simulink model "kundur_sync"  (R2023b)
settings: Solver=ode23tb  StartTime=0.0  StopTime=200  MaxStep=1/60  RelTol=1e-3
InitFcn:
  | SolarInverter_Params();
values from neighbouring files (symbols this model uses):
  Fnom = 60    [SolarInverter_Params.m]
  Pnom = 900e6    (= 900000000)    [SolarInverter_Params.m]
  reec_dbd1 = -0.1    [SolarInverter_Params.m]
  reec_dbd2 = 0.1    [SolarInverter_Params.m]
  reec_dPmax = 0.1    [SolarInverter_Params.m]
  reec_dPmin = -0.1    [SolarInverter_Params.m]
  reec_Imax = 1    [SolarInverter_Params.m]
  reec_Iqhl = 1.0    (= 1)    [SolarInverter_Params.m]
  reec_Iqll = -0.4    [SolarInverter_Params.m]
  reec_Kqi = 0.0    (= 0)    [SolarInverter_Params.m]
  reec_Kqp = 0    [SolarInverter_Params.m]
  reec_Kvi = 0.0    (= 0)    [SolarInverter_Params.m]
  reec_Kvp = 0.1    [SolarInverter_Params.m]
  reec_Pmax = 1.0    (= 1)    [SolarInverter_Params.m]
  reec_Pmin = 0    [SolarInverter_Params.m]
  reec_Qmax = 0.435    [SolarInverter_Params.m]
  reec_Qmin = -0.435    [SolarInverter_Params.m]
  reec_Tiq = 0.02    [SolarInverter_Params.m]
  reec_Tp = 0.02    [SolarInverter_Params.m]
  reec_Tpord = 0.1    [SolarInverter_Params.m]
  reec_Trv = 0.01    [SolarInverter_Params.m]
  reec_Vdip = 0.9    [SolarInverter_Params.m]
  reec_Vmax = 1.10    (= 1.1)    [SolarInverter_Params.m]
  reec_Vmin = 0.9    [SolarInverter_Params.m]
  reec_Vup = 1.15    [SolarInverter_Params.m]
  regc_Brkpt = 0.9    [SolarInverter_Params.m]
  regc_Iolim = -1.2    [SolarInverter_Params.m]
  regc_Iqrmax = 999.9    [SolarInverter_Params.m]
  regc_Iqrmin = -999.9    [SolarInverter_Params.m]
  regc_Ivpnt0 = 0.4    [SolarInverter_Params.m]
  regc_Ivpnt1 = 0.8    [SolarInverter_Params.m]
  regc_Khv = 0.0    (= 0)    [SolarInverter_Params.m]
  regc_Lvpl1 = 1.0    (= 1)    [SolarInverter_Params.m]
  regc_Lvplsw = 0    [SolarInverter_Params.m]
  regc_rrpwr = 10    [SolarInverter_Params.m]
  regc_Tfltr = 0.02    [SolarInverter_Params.m]
  regc_Tg = 0.1    [SolarInverter_Params.m]
  regc_Volim = 1.1    [SolarInverter_Params.m]
  regc_Zerox = 0.5    [SolarInverter_Params.m]
  repc_db1 = 0    [SolarInverter_Params.m]
  repc_Ddn = 20    [SolarInverter_Params.m]
  repc_Dup = 0    [SolarInverter_Params.m]
  repc_emax = 999    [SolarInverter_Params.m]
  repc_emin = -999    [SolarInverter_Params.m]
  repc_fdbd1 = 0.01*0    (= 0)    [SolarInverter_Params.m]
  repc_fdbd2 = -0.01*0    (= 0)    [SolarInverter_Params.m]
  repc_femax = 999    [SolarInverter_Params.m]
  repc_femin = -999    [SolarInverter_Params.m]
  repc_Kc = 0.05    [SolarInverter_Params.m]
  repc_Ki = 1.8    [SolarInverter_Params.m]
  repc_Kig = 0.5    [SolarInverter_Params.m]
  repc_Kp = 0.6    [SolarInverter_Params.m]
  repc_Kpg = 0.1    [SolarInverter_Params.m]
  repc_Pmax = 1    [SolarInverter_Params.m]
  repc_Pmin = 0    [SolarInverter_Params.m]
  repc_Qmax = 0.435    [SolarInverter_Params.m]
  repc_Qmin = -0.435    [SolarInverter_Params.m]
  repc_Rc = 0    [SolarInverter_Params.m]
  repc_Tfltr = 0.02    [SolarInverter_Params.m]
  repc_Tft = 0.5    [SolarInverter_Params.m]
  repc_Tfv = 0.8    [SolarInverter_Params.m]
  repc_Tlag = 0.2    [SolarInverter_Params.m]
  repc_Tp = 0.25    [SolarInverter_Params.m]
  repc_Vfrz = 0.7    [SolarInverter_Params.m]
  repc_Xc = 0    [SolarInverter_Params.m]
  Vnom = 230e3    (= 230000)    [SolarInverter_Params.m]
undefined symbols (not defined in the file or in its folder): D1, Delta, gcbh, j, k_fault, k_pulse, sps_rtmsupport
libraries: powerlib_extras x24, simulink x13, spsLoadFlowBusLib x12, spsThreePhaseVIMeasurementLib x11, spsThreePhasePISectionLineLib x8, spsThreePhaseTransformerTwoWindingsLib x5, spsThreePhaseParallelRLCLoadLib x4, spsSynchronousMachinepuStandardLib x4, spsExcitationSystemLib x4, spsSteamTurbineandGovernorLib x4, spsGenericPowerSystemStabilizerLib x4, spsControlledCurrentSourceLib x2
(part 1 of 3)
settings Model: Creator=jlesage  LastModifiedBy=shura
settings SolverCC: ZeroCrossAlgorithm=Adaptive
settings DataIOCC: InitialState=getstatestruct(opreport)  SaveOutput=off  SignalLogging=off  DSMLogging=off  SaveTime=off  ReturnWorkspaceOutputs=off
settings DebuggingCC: IgnoredZcDiagnostic=none
settings ModelReferenceCC: EnableRefExpFcnMdlSchedulingChecks=on
settings SFSimCC: CustomCodeUndefinedFunction=UseInterfaceOnly
settings SimscapeCC: SimscapeNormalizeSystem=off

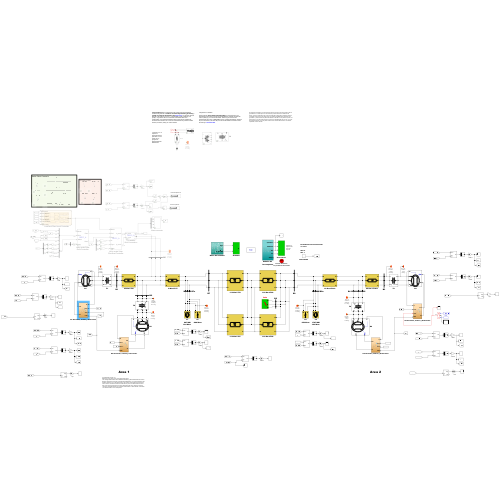
[thumbnail: Simulink's stored preview of the top-level diagram]
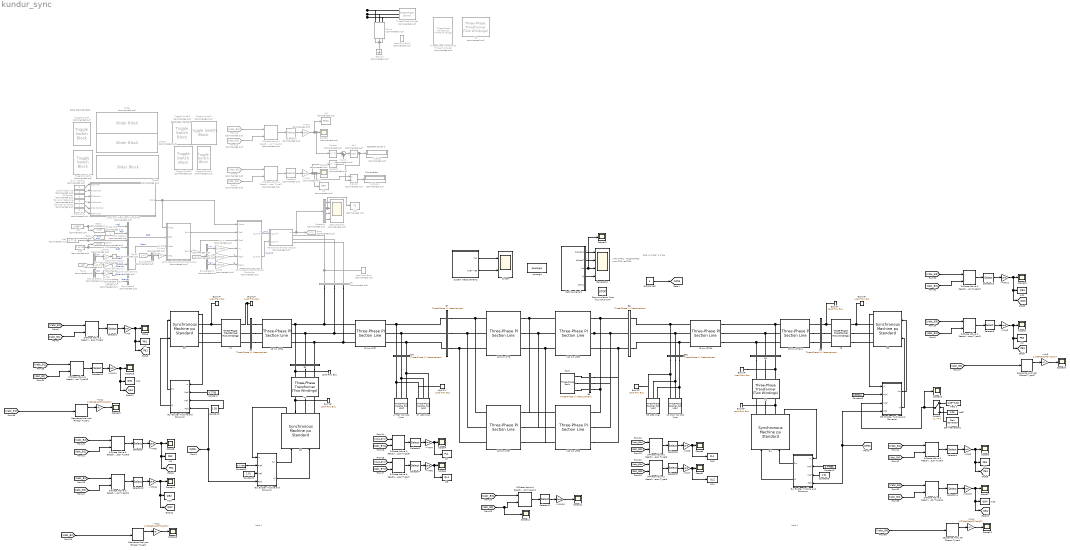
== system kundur_sync ==
  note: Solar Plant Controls
  note: Secondary Controls
  note: yellow=G1,
      | magenta=G2,
      | cyan=G3,
      | red=G4
  note: Area 2
  note: Area 1
  note: PSS: 0 = OFF, 1 = ON
  note: Power factor
  note: Apparent power S
  ->MW{,2..8,10..14} (13 alike) : Gain  Gain=1e-6  SaturateOnIntegerOverflow=on  OutDataTypeStr=Inherit: Same as input  ParamDataTypeStr=Inherit: Same as input
  ->MW1 : Gain  Commented=on  Gain=1e-6  SaturateOnIntegerOverflow=on  OutDataTypeStr=Inherit: Same as input  ParamDataTypeStr=Inherit: Same as input
  ->MW9 : Gain  Commented=on  Gain=1e-6  SaturateOnIntegerOverflow=on  OutDataTypeStr=Inherit: Same as input  ParamDataTypeStr=Inherit: Same as input
  ->pu{1..4} (4 alike) : Gain  Gain=1/(230e3/sqrt(3)*sqrt(2))  SaturateOnIntegerOverflow=on  OutDataTypeStr=Inherit: Same as input  ParamDataTypeStr=Inherit: Same as input
  10 Km LT67 : spsThreePhasePISectionLineLib/Three-Phase PI Section Line  LConnTagsString=a|b|c  RConnTagsString=A|B|C  Length=10  Frequency=60  Resistances=[0.0001*529 1.61]  Inductances=[0.001*529/(377) 0.0061]  Capacitances=[0.00175/529/(377) 5.2489e-9]
  10 Km LT910 : spsThreePhasePISectionLineLib/Three-Phase PI Section Line  LConnTagsString=a|b|c  RConnTagsString=A|B|C  Length=10  Frequency=60  Resistances=[0.0001*529 1.61]  Inductances=[0.001*529/(377) 0.0061]  Capacitances=[0.00175/529/(377) 5.2489e-9]
  110 Km LT{78,87,89,98} (4 alike) : spsThreePhasePISectionLineLib/Three-Phase PI Section Line  LConnTagsString=a|b|c  RConnTagsString=A|B|C  Length=110  Frequency=60  Resistances=[0.0001*529 1.61]  Inductances=[0.001*529/(377) 0.0061]  Capacitances=[0.00175/529/(377) 5.2489e-9]
  25 Km LT1011 : spsThreePhasePISectionLineLib/Three-Phase PI Section Line  LConnTagsString=a|b|c  RConnTagsString=A|B|C  Length=25  Frequency=60  Resistances=[0.0001*529 1.61]  Inductances=[0.001*529/(377) 0.0061]  Capacitances=[0.00175/529/(377) 5.2489e-9]
  25 Km LT56 : spsThreePhasePISectionLineLib/Three-Phase PI Section Line  LConnTagsString=a|b|c  RConnTagsString=A|B|C  Length=25  Frequency=60  Resistances=[0.0001*529 1.61]  Inductances=[0.001*529/(377) 0.0061]  Capacitances=[0.00175/529/(377) 5.2489e-9]
  3-Phase Active & Reactive Power (Phasor Type){1,3..9,11..15} (13 alike) : powerlib_extras/Phasor Library/3-Phase Active & Reactive Power (Phasor Type)
  3-Phase Active & Reactive Power (Phasor Type)10 : powerlib_extras/Phasor Library/3-Phase Active & Reactive Power (Phasor Type)  Commented=on
  3-Phase Active & Reactive Power (Phasor Type)2 : powerlib_extras/Phasor Library/3-Phase Active & Reactive Power (Phasor Type)  Commented=on
  B1 : spsThreePhaseVIMeasurementLib/Three-Phase V-I Measurement  VoltageMeasurement=phase-to-ground  SetLabelV=on  LabelV=Vabc_B1  Vpu=off  VpuLL=off  CurrentMeasurement=yes  SetLabelI=on  LabelI=Iabc_B1  Ipu=off  Pbase=100e6  Vbase=500e3  OutputType=Complex  PhasorSimulation=on  PSBequivalent=0
  B2 : spsThreePhaseVIMeasurementLib/Three-Phase V-I Measurement  VoltageMeasurement=phase-to-ground  SetLabelV=on  LabelV=Vabc_B2  Vpu=off  VpuLL=off  CurrentMeasurement=yes  SetLabelI=on  LabelI=Iabc_B2  Ipu=off  Pbase=100e6  Vbase=500e3  OutputType=Complex  PhasorSimulation=on  PSBequivalent=0
  B3 : spsThreePhaseVIMeasurementLib/Three-Phase V-I Measurement  VoltageMeasurement=phase-to-ground  SetLabelV=on  LabelV=Vabc_B3  Vpu=off  VpuLL=off  CurrentMeasurement=yes  SetLabelI=on  LabelI=Iabc_B3  Ipu=off  Pbase=100e6  Vbase=500e3  OutputType=Complex  PhasorSimulation=on  PSBequivalent=0
  B4 : spsThreePhaseVIMeasurementLib/Three-Phase V-I Measurement  VoltageMeasurement=phase-to-ground  SetLabelV=on  LabelV=Vabc_B4  Vpu=off  VpuLL=off  CurrentMeasurement=yes  SetLabelI=on  LabelI=Iabc_B4  Ipu=off  Pbase=100e6  Vbase=500e3  OutputType=Complex  PhasorSimulation=on  PSBequivalent=0
  B5 : spsThreePhaseVIMeasurementLib/Three-Phase V-I Measurement  Commented=on  VoltageMeasurement=phase-to-ground  SetLabelV=on  LabelV=Vabc_B5  Vpu=off  VpuLL=off  CurrentMeasurement=yes  SetLabelI=on  LabelI=Iabc_B5  Ipu=off  Pbase=100e6  Vbase=500e3  OutputType=Complex  PhasorSimulation=on  PSBequivalent=0
  B6 : spsThreePhaseVIMeasurementLib/Three-Phase V-I Measurement  VoltageMeasurement=phase-to-ground  SetLabelV=on  LabelV=Vabc_B8  Vpu=off  VpuLL=off  CurrentMeasurement=yes  SetLabelI=on  LabelI=Iabc_B8  Ipu=off  Pbase=100e6  Vbase=500e3  OutputType=Complex  PhasorSimulation=on  PSBequivalent=0
  B7 : spsThreePhaseVIMeasurementLib/Three-Phase V-I Measurement  VoltageMeasurement=phase-to-ground  SetLabelV=on  LabelV=Vabc_B7  Vpu=off  VpuLL=off  CurrentMeasurement=yes  SetLabelI=on  LabelI=Iabc_B7  Ipu=off  Pbase=100e6  Vbase=500e3  OutputType=Complex  PhasorSimulation=on  PSBequivalent=0
  B7c : spsThreePhaseVIMeasurementLib/Three-Phase V-I Measurement  VoltageMeasurement=phase-to-ground  SetLabelV=on  LabelV=Vabc_B7c  Vpu=off  VpuLL=off  CurrentMeasurement=yes  SetLabelI=on  LabelI=Iabc_B7c  Ipu=off  Pbase=100e6  Vbase=500e3  OutputType=Complex  PhasorSimulation=on  PSBequivalent=0
  B9 : spsThreePhaseVIMeasurementLib/Three-Phase V-I Measurement  VoltageMeasurement=phase-to-ground  SetLabelV=on  LabelV=Vabc_B9  Vpu=off  VpuLL=off  CurrentMeasurement=yes  SetLabelI=on  LabelI=Iabc_B9  Ipu=off  Pbase=100e6  Vbase=500e3  OutputType=Complex  PhasorSimulation=on  PSBequivalent=0
  B9c : spsThreePhaseVIMeasurementLib/Three-Phase V-I Measurement  VoltageMeasurement=phase-to-ground  SetLabelV=on  LabelV=Vabc_B9c  Vpu=off  VpuLL=off  CurrentMeasurement=yes  SetLabelI=on  LabelI=Iabc_B9c  Ipu=off  Pbase=100e6  Vbase=500e3  OutputType=Complex  PhasorSimulation=on  PSBequivalent=0
  Bus Creator1 : BusCreator  Commented=on  Inputs=4
  Bus Creator2 : BusCreator  Commented=on  Inputs=4
  Bus Selector1 : BusSelector  Commented=on  OutputSignals=V,P,Q
  Bus Selector2 : BusSelector  Commented=on  OutputSignals=F,P,Q
  Bus Selector3 : BusSelector  Commented=on  OutputSignals=V
  Bus*13* : spsLoadFlowBusLib/Load Flow Bus  LConnTagsString=a  Phases=single  Connectors=on one side  ID=Bus*13*  Vbase=230000  Vref=1  Vangle=0  VLF=1.007  VLFb=1  VLFc=1  angleLF=43.46  angleLFb=0  angleLFc=0
  Bus*14* : spsLoadFlowBusLib/Load Flow Bus  LConnTagsString=a  Phases=single  Connectors=on one side  ID=Bus*14*  Vbase=20000  Vref=1.03  Vangle=20.2  VLF=1.03  VLFb=1  VLFc=1  angleLF=19.92  angleLFb=0  angleLFc=0
  Bus*16* : spsLoadFlowBusLib/Load Flow Bus  LConnTagsString=a  Phases=single  Connectors=on one side  ID=Bus*16*  Vbase=20000  Vref=1.01  Vangle=10.5  VLF=1.01  VLFb=1  VLFc=1  angleLF=10.17  angleLFb=0  angleLFc=0
  Bus*17* : spsLoadFlowBusLib/Load Flow Bus  LConnTagsString=a  Phases=single  Connectors=on one side  ID=Bus*17*  Vbase=230000  Vref=1  Vangle=0  VLF=1.009  VLFb=1  VLFc=1  angleLF=16.59  angleLFb=0  angleLFc=0
  Bus*18* : spsLoadFlowBusLib/Load Flow Bus  LConnTagsString=a  Phases=single  Connectors=on one side  ID=Bus*18*  Vbase=20000  Vref=1.03  Vangle=-6.8  VLF=1.03  VLFb=1  VLFc=1  angleLF=-6.8  angleLFb=0  angleLFc=0
  Bus*19* : spsLoadFlowBusLib/Load Flow Bus  LConnTagsString=a  Phases=single  Connectors=on one side  ID=Bus*19*  Vbase=230000  Vref=1  Vangle=0  VLF=0.9863  VLFb=1  VLFc=1  angleLF=6.317  angleLFb=0  angleLFc=0
  Bus*20* : spsLoadFlowBusLib/Load Flow Bus  LConnTagsString=a  Phases=single  Connectors=on one side  ID=Bus*20*  Vbase=20000  Vref=1.01  Vangle=-17  VLF=1.01  VLFb=1  VLFc=1  angleLF=-16.96  angleLFb=0  angleLFc=0
  Bus*21* : spsLoadFlowBusLib/Load Flow Bus  LConnTagsString=a  Phases=single  Connectors=on one side  ID=Bus*21*  Vbase=230000  Vref=1  Vangle=0  VLF=0.9654  VLFb=1  VLFc=1  angleLF=25.05  angleLFb=0  angleLFc=0
  Bus*22* : spsLoadFlowBusLib/Load Flow Bus  LConnTagsString=a  Phases=single  Connectors=on one side  ID=Bus*22*  Vbase=230000  Vref=1  Vangle=0  VLF=0.9765  VLFb=1  VLFc=1  angleLF=-2.038  angleLFb=0  angleLFc=0
  C7 -200 Mvar : spsThreePhaseParallelRLCLoadLib/Three-Phase Parallel RLC Load  LConnTagsString=A|B|C  Configuration=Y (grounded)  NominalVoltage=(230000)*0.965432  Vabc=[1e3 1e3 1e3]  Vabcp=[1e3 1e3 1e3]  NominalFrequency=60  UnbalancedPower=off  ActivePower=0  InductivePower=0  CapacitivePower=200000000  Pabc=[10e3 9e3 11e3]  QLabc=[100 90 110]  QCabc=[100 90 110]  Pabcp=[10e3 9e3 11e3]  QLabcp=[100 90 110]  QCabcp=[100 90 110]  Measurements=None  LoadType=constant PQ
  C9 -350 Mvar : spsThreePhaseParallelRLCLoadLib/Three-Phase Parallel RLC Load  LConnTagsString=A|B|C  Configuration=Y (grounded)  NominalVoltage=(230000)*0.976525  Vabc=[1e3 1e3 1e3]  Vabcp=[1e3 1e3 1e3]  NominalFrequency=60  UnbalancedPower=off  ActivePower=0  InductivePower=0  CapacitivePower=350000000  Pabc=[10e3 9e3 11e3]  QLabc=[100 90 110]  QCabc=[100 90 110]  Pabcp=[10e3 9e3 11e3]  QLabcp=[100 90 110]  QCabcp=[100 90 110]  Measurements=None  LoadType=constant PQ
  Constant : Constant  Value=0.7793
  Constant1 : Constant  Value=1.03
  Constant13 : Constant  Commented=on
  Constant14 : Constant  Commented=on  Value=0
  Constant2 : Constant  Value=0.77941
  Constant3 : Constant  Value=1.01
  Constant5 : Constant  Value=0.80012
  Constant6 : Constant  Value=1.01
  Constant7 : Constant  Value=0.77936
  Coordinated V/Q : Constant  Commented=on
  System measurements : Subsystem
  Stop simulation (loss of synchronism) : Stop
  Display : Display  Commented=on
  Display1 : Display  Commented=on
  Fault : spsThreePhaseFaultLib/Three-Phase Fault  InitialStates=0  FaultA=on  FaultB=on  FaultC=on  GroundFault=on  SwitchTimes=[150 150+12/60]*k_fault  External=off  SwitchStatus=NaN  FaultResistance=0.1  GroundResistance=0.1  SnubberResistance=inf  SnubberCapacitance=0  Measurements=None
  From : From  Commented=on  GotoTag=m
  From1 : From  Commented=on  GotoTag=m
  From2 : From  Commented=on  GotoTag=m
  From23 : From  Commented=on  GotoTag=Iabc_B5  TagVisibility=global
      settings: CloseFcn=tagdialog Close
  From24 : From  Commented=on  GotoTag=Vabc_B5  TagVisibility=global
      settings: CloseFcn=tagdialog Close
  From7 : From  Commented=on  GotoTag=Iabc_B5  TagVisibility=global
      settings: CloseFcn=tagdialog Close
  From8 : From  Commented=on  GotoTag=Vabc_B5  TagVisibility=global
      settings: CloseFcn=tagdialog Close
  G1 : spsSynchronousMachinepuStandardLib/Synchronous Machine pu Standard  PresetModel=No  MechanicalLoad=Mechanical power Pm  ShowDetailedParameters=on  RotorType=Round  Units=per unit standard parameters  MeasurementBus=off  NominalParameters=[900E6 20E3 60]  Reactances1=[ 1.8, 0.3, 0.25, 1.7, 0.55, 0.25, 0.2 ]  Reactances2=[2.24 0.17 0.12 1.02 0.13 0.08]  dAxisTimeConstants=Open-circuit  qAxisTimeConstants=Open-circuit  TimeConstants1="[ 4.4849  0.0681  0.1  ]"  TimeConstants2=[ 8.0, 0.03, 0.4, 0.05 ]  TimeConstants3="[  4.49  0.0681  0.0513  ]"  TimeConstants4=[ 8.0, 0.03, 0.3371, 0.0295 ]  TimeConstants5=[ 1.01, 0.053, 0.1 ]  TimeConstants6=[ 1.3201, 0.023, 1.0, 0.07 ]  TimeConstants7=[0.012 0.003 0.003]  TimeConstants8=[ 1.3201, 0.0231, 0.3371, 0.0295 ]  StatorResistance=0.0025  Mechanical=[6.5 0 1]  PolePairs=20  InitialConditions=[0 -26.7419 0.779382 0.779382 0.779382 5.5866 -114.413 125.587 1.9356]  SetSaturation=off  Saturation=[0.6404,0.7127,0.8441,0.9214,0.9956,1.082,1.19,1.316,1.457;0.7,0.7698,0.8872,0.9466,0.9969,1.046,1.1,1.151,1.201]  LoadFlowParameters=[1 700000000 0 0 0]  TsPowergui=0  TsBlock=-1  IterativeModel=Trapezoidal non iterative  IterativeDiscreteModel=Trapezoidal non iterative  BusType=PV  Pref=700000000  Qref=0  Qmin=-Inf  Qmax=Inf  PLF=0  QLF=0
  "G1: Exciter, Turbine and Governor" : Subsystem
  G2 : spsSynchronousMachinepuStandardLib/Synchronous Machine pu Standard  PresetModel=No  MechanicalLoad=Mechanical power Pm  ShowDetailedParameters=on  RotorType=Round  Units=per unit standard parameters  MeasurementBus=off  NominalParameters=[900E6 20E3 60]  Reactances1=[ 1.8, 0.3, 0.25, 1.7, 0.55, 0.25, 0.2 ]  Reactances2=[2.24 0.17 0.12 1.02 0.13 0.08]  dAxisTimeConstants=Open-circuit  qAxisTimeConstants=Open-circuit  TimeConstants1="[ 4.4849  0.0681  0.1  ]"  TimeConstants2=[ 8.0, 0.03, 0.4, 0.05 ]  TimeConstants3="[  4.49  0.0681  0.0513  ]"  TimeConstants4=[ 8.0, 0.03, 0.3371, 0.0295 ]  TimeConstants5=[ 1.01, 0.053, 0.1 ]  TimeConstants6=[ 1.3201, 0.023, 1.0, 0.07 ]  TimeConstants7=[0.012 0.003 0.003]  TimeConstants8=[ 1.3201, 0.0231, 0.3371, 0.0295 ]  StatorResistance=0.0025  Mechanical=[6.5 0 1]  PolePairs=20  InitialConditions=[0 -37.2189 0.807096 0.807096 0.807096 -7.24574 -127.246 112.754 2.00287]  SetSaturation=off  Saturation=[0.6404,0.7127,0.8441,0.9214,0.9956,1.082,1.19,1.316,1.457;0.7,0.7698,0.8872,0.9466,0.9969,1.046,1.1,1.151,1.201]  LoadFlowParameters=[1 700000000 0 0 0]  TsPowergui=0  TsBlock=-1  IterativeModel=Trapezoidal non iterative  IterativeDiscreteModel=Trapezoidal non iterative  BusType=PV  Pref=700000000  Qref=0  Qmin=-Inf  Qmax=Inf  PLF=0  QLF=0
  "G2: Exciter, Turbine and Governor" : Subsystem
  G3 : spsSynchronousMachinepuStandardLib/Synchronous Machine pu Standard  PresetModel=No  MechanicalLoad=Mechanical power Pm  ShowDetailedParameters=on  RotorType=Round  Units=per unit standard parameters  MeasurementBus=off  NominalParameters=[900E6 20E3 60]  Reactances1=[ 1.8, 0.3, 0.25, 1.7, 0.55, 0.25, 0.2 ]  Reactances2=[2.24 0.17 0.12 1.02 0.13 0.08]  dAxisTimeConstants=Open-circuit  qAxisTimeConstants=Open-circuit  TimeConstants1="[ 4.4849  0.0681  0.1  ]"  TimeConstants2=[ 8.0, 0.03, 0.4, 0.05 ]  TimeConstants3="[  4.49  0.0681  0.0513  ]"  TimeConstants4=[ 8.0, 0.03, 0.3371, 0.0295 ]  TimeConstants5=[ 1.01, 0.053, 0.1 ]  TimeConstants6=[ 1.3201, 0.023, 1.0, 0.07 ]  TimeConstants7=[0.012 0.003 0.003]  TimeConstants8=[ 1.3201, 0.0231, 0.3371, 0.0295 ]  StatorResistance=0.0025  Mechanical=[6.175 0 1]  PolePairs=20  InitialConditions=[0 -52.3113 0.79634 0.79634 0.79634 -20.0073 -140.007 99.9927 1.94741]  SetSaturation=off  Saturation=[0.6404,0.7127,0.8441,0.9214,0.9956,1.082,1.19,1.316,1.457;0.7,0.7698,0.8872,0.9466,0.9969,1.046,1.1,1.151,1.201]  LoadFlowParameters=[2 719000000 0 -6.8 0]  TsPowergui=0  TsBlock=-1  IterativeModel=Trapezoidal non iterative  IterativeDiscreteModel=Trapezoidal non iterative  BusType=swing  Pref=Inf  Qref=0  Qmin=-Inf  Qmax=Inf  PLF=0  QLF=0
  "G3: Exciter, Turbine and Governor" : Subsystem
  G4 : spsSynchronousMachinepuStandardLib/Synchronous Machine pu Standard  PresetModel=No  MechanicalLoad=Mechanical power Pm  ShowDetailedParameters=on  RotorType=Round  Units=per unit standard parameters  MeasurementBus=off  NominalParameters=[900E6 20E3 60]  Reactances1=[ 1.8, 0.3, 0.25, 1.7, 0.55, 0.25, 0.2 ]  Reactances2=[2.24 0.17 0.12 1.02 0.13 0.08]  dAxisTimeConstants=Open-circuit  qAxisTimeConstants=Open-circuit  TimeConstants1="[ 4.4849  0.0681  0.1  ]"  TimeConstants2=[ 8.0, 0.03, 0.4, 0.05 ]  TimeConstants3="[  4.49  0.0681  0.0513  ]"  TimeConstants4=[ 8.0, 0.03, 0.3371, 0.0295 ]  TimeConstants5=[ 1.01, 0.053, 0.1 ]  TimeConstants6=[ 1.3201, 0.023, 1.0, 0.07 ]  TimeConstants7=[0.012 0.003 0.003]  TimeConstants8=[ 1.3201, 0.0231, 0.3371, 0.0295 ]  StatorResistance=0.0025  Mechanical=[6.175 0 1]  PolePairs=20  InitialConditions=[0 -62.9983 0.796384 0.796384 0.796384 -31.7259 -151.726 88.2741 1.95328]  SetSaturation=off  Saturation=[0.6404,0.7127,0.8441,0.9214,0.9956,1.082,1.19,1.316,1.457;0.7,0.7698,0.8872,0.9466,0.9969,1.046,1.1,1.151,1.201]  LoadFlowParameters=[1 700000000 0 0 0]  TsPowergui=0  TsBlock=-1  IterativeModel=Trapezoidal non iterative  IterativeDiscreteModel=Trapezoidal non iterative  BusType=PV  Pref=700000000  Qref=0  Qmin=-Inf  Qmax=Inf  PLF=0  QLF=0
  "G4: Exciter, Turbine and Governor" : Subsystem
  Generators : Scope  NumInputPorts=4
  Goto : Goto  Commented=on  GotoTag=m
  Goto1 : Goto  Commented=on  GotoTag=Pref  TagVisibility=global
  Goto2 : Goto  Commented=on  GotoTag=Vref  TagVisibility=global
  Goto3 : Goto  Commented=on  GotoTag=Qref  TagVisibility=global
  Governor Response : Constant  Commented=on
  Ground : spsGroundLib/Ground  Commented=on  LConnTagsString=a
  L7 967 MW 100 Mvar : spsThreePhaseParallelRLCLoadLib/Three-Phase Parallel RLC Load  LConnTagsString=A|B|C  Configuration=Y (grounded)  NominalVoltage=(230000)*0.965432  Vabc=[1e3 1e3 1e3]  Vabcp=[1e3 1e3 1e3]  NominalFrequency=60  UnbalancedPower=off  ActivePower=967000000  InductivePower=100000000  CapacitivePower=0  Pabc=[10e3 9e3 11e3]  QLabc=[100 90 110]  QCabc=[100 90 110]  Pabcp=[10e3 9e3 11e3]  QLabcp=[100 90 110]  QCabcp=[100 90 110]  Measurements=None  LoadType=constant PQ
  L9 1767 MW 100 Mvar : spsThreePhaseParallelRLCLoadLib/Three-Phase Parallel RLC Load  LConnTagsString=A|B|C  Configuration=Y (grounded)  NominalVoltage=(230000)*0.976525  Vabc=[1e3 1e3 1e3]  Vabcp=[1e3 1e3 1e3]  NominalFrequency=60  UnbalancedPower=off  ActivePower=1767000000  InductivePower=100000000  CapacitivePower=0  Pabc=[10e3 9e3 11e3]  QLabc=[100 90 110]  QCabc=[100 90 110]  Pabcp=[10e3 9e3 11e3]  QLabcp=[100 90 110]  QCabcp=[100 90 110]  Measurements=None  LoadType=constant PQ
  Load Flow Bus : spsLoadFlowBusLib/Load Flow Bus  LConnTagsString=a  Phases=single  Connectors=on one side  ID=BUS_1  Vbase=230000  Vref=1  Vangle=0  VLF=0.9806  VLFb=1  VLFc=1  angleLF=33.41  angleLFb=0  angleLFc=0
  Load Flow Bus1 : spsLoadFlowBusLib/Load Flow Bus  Commented=on  LConnTagsString=a  Phases=single  Connectors=on one side  ID=BUS_19  Vbase=20000  Vref=1.01  Vangle=10.17  VLF=0.9613  VLFb=1  VLFc=1  angleLF=-36.41  angleLFb=0  angleLFc=0
  Load Flow Bus2 : spsLoadFlowBusLib/Load Flow Bus  Commented=on  LConnTagsString=a  Phases=single  Connectors=on one side  ID=BUS_20  Vbase=230000  Vref=0.9807  Vangle=33.41  VLF=0.9616  VLFb=1  VLFc=1  angleLF=-36.39  angleLFb=0  angleLFc=0
  Local and Plant Level Controller : Stateflow chart  Commented=on  InitFcn=|  TreatAsAtomicUnit=on
      | BusElement(1) = Simulink.BusElement;
      | BusElement(1).Name = 'QFlag';
      | BusElement(1).Dimensions = 1;
      | BusElement(1).DimensionsMode = 'Fixed';
      | BusElement(1).DataType = 'double';
      | BusElement(1).Complexity = 'real';
      | 
      | BusElement(2) = Simulink.BusElement;
      | BusElement(2).Name = 'VFlag';
      | BusElement(2).Dimensions = 1;
      | BusElement(2).DimensionsMode = 'Fixed';
      | BusElement(2).DataType = 'double';
      | BusElement(2).Complexity = 'real';
      | 
      | BusElement(3) = Simulink.BusElement;
      | BusElement(3).Name = 'PfFlag';
      | BusElement(3).Dimensions = 1;
      | BusElement(3).DimensionsMode = 'Fixed';
      | BusElement(3).DataType = 'double';
      | BusElement(3).Complexity = 'real';
      | 
      | BusElement(4) = Simulink.BusElement;
      | BusElement(4).Name = 'PqFlag';
      | BusElement(4).Dimensions = 1;
      | BusElement(4).DimensionsMode = 'Fixed';
      | BusElement(4).DataType = 'double';
      | BusElement(4).Complexity = 'real';
      | 
      | BusElement(5) = Simulink.BusElement;
      | BusElement(5).Name = 'VcompFlag';
      | BusElement(5).Dimensions = 1;
      | BusElement(5).DimensionsMode = 'Fixed';
      | BusElement(5).DataType = 'double';
      | BusElement(5).Complexity = 'real';
      | 
      | BusElement(6) = Simulink.BusElement;
      | BusElement(6).Name = 'RefFlag';
      | BusElement(6).Dimensions = 1;
      | BusElement(6).DimensionsMode = 'Fixed';
      | BusElement(6).DataType = 'double';
      | BusElement(6).Complexity = 'real';
      | 
      | BusElement(7) = Simulink.BusElement;
      | BusElement(7).Name = 'FrqFlag';
      | BusElement(7).Dimensions = 1;
      | BusElement(7).DimensionsMode = 'Fixed';
      | BusElement(7).DataType = 'double';
      | BusElement(7).Complexity = 'real';
      | 
      | Mode = Simulink.Bus;
      | Mode.Elements = BusElement;
      | 
      | clearvars BusElement
  Measurements : Scope  Commented=on  NumInputPorts=4
  OFF/ON PSS : Constant  SampleTime=1/60
  P/Q Priority : Constant  Commented=on  Value=0
  PF Control : Constant  Commented=on
  Plant-Level Control : Constant  Commented=on
  Pref : Constant  Commented=on  Value=0.7778
  Product : Product  Commented=on  Inputs=*/
  Q or V Control : Constant  Commented=on
  Qref : Constant  Commented=on  Value=0.10795
  Renewable Grid-Connection : Subsystem  Commented=on  mask(Renewable Energy Grid Connection (REGC_A)){Tfltr=regc_Tfltr, Lvpl1=regc_Lvpl1, Zerox=regc_Zerox, Brkpt=regc_Brkpt, Lvplsw=regc_Lvplsw, rrpwr=regc_rrpwr, Tg=regc_Tg, Volim=regc_Volim, Iolim=regc_Iolim, Khv=regc_Khv, Ivpnt0=regc_Ivpnt0, Ivpnt1=regc_Ivpnt1, Iqrmax=regc_Iqrmax, Iqrmin=regc_Iqrmin}
      mask prompts: Tfltr "Tfltr - Terminal Voltage Filter [s]"; Lvpl1 "Lvpl1 - LVPL Gain Breakpoint [pu]"; Zerox "Zerox - LVPL Zero Crossing [pu]"; Brkpt "Brkpt - LVPL Breakpoint [pu]"; Lvplsw "Lvplsw - Low Voltage Power Logic [Enable (1) or Disable (0)]"; rrpwr "rrpwr - Active Current up-ramp rater limit [pu/s]"; Tg "Tg - Inverter Current Lag Time [s]"; Volim "Volim - Voltage Limit Clap Logic [pu]"; Iolim "Iolim - Current Limit for Clap Logic [pu]"; Khv "Khv - High Voltage Clap Logic Factor"; Ivpnt0 "Ivpnt0 - Low voltage current breakpoint [pu]"; Ivpnt1 "Ivpnt1 - Low voltage current breakpoint [pu]"; Iqrmax "Iqrmax - Maximum rate of change [pu/s]"; Iqrmin "Iqrmin - Minimum rate of change [pu/s]"
      mask help: REGC_A module, used to represent the Generator/Converter (inverter) interface with the grid. It processes the real and reactive current command and outputs of real and reactive current injection into the grid model.
      mask Display: color('blue');disp('REGC_A')
  Scope{,2..8,10..21} (20 alike) : Scope
  Scope1 : Scope  Commented=on
  Scope9 : Scope  Commented=on
  Selection : Subsystem  Commented=on
  Selector{1,3..6,9,11} (7 alike) : Selector  InputPortWidth=2  IndexOptions=Index vector (dialog)  Indices=1  OutputSizes=1
  Selector10 : Selector  Commented=on  InputPortWidth=2  IndexOptions=Index vector (dialog)  Indices=2  OutputSizes=1
  Selector{7..8,12..15} (6 alike) : Selector  InputPortWidth=2  IndexOptions=Index vector (dialog)  Indices=2  OutputSizes=1
  Selector2 : Selector  Commented=on  InputPortWidth=2  IndexOptions=Index vector (dialog)  Indices=1  OutputSizes=1
  Sequence Analyzer (Phasor Type){1..4} (4 alike) : powerlib_extras/Phasor Library/Sequence Analyzer (Phasor Type)  seq=Positive
  Machine signals : Subsystem
  Shunt : spsThreePhaseSeriesRLCBranchLib/Three-Phase Series RLC Branch  Commented=on  LConnTagsString=A|B|C  RConnTagsString=A|B|C  BranchType=R  Resistance=1e9  Inductance=0  Capacitance=1e-6  Measurements=None
  Signal Conversion : SignalConversion  Commented=on  OverrideOpt=off
  Signal Conversion1 : SignalConversion  Commented=on  OverrideOpt=off
  Signal Conversion2 : SignalConversion  Commented=on  OverrideOpt=off
  System : Scope  NumInputPorts=2
  Slider : SliderBlock  Commented=on  ScaleMin=0.94999999999999996  ScaleMax=1.05
  Slider1 : SliderBlock  Commented=on  ScaleMax=1  TickInterval=0.25
  Slider2 : SliderBlock  Commented=on  ScaleMin=-1  ScaleMax=1
  Sqrt : Sqrt  Commented=on
  Square : Math  Commented=on  Operator=square  SignedPower=on
  Square1 : Math  Commented=on  Operator=square  SignedPower=on
  Stair Generator1 : spsStairGeneratorLib/Stair Generator  t=[0 150 150+6/60]*k_pulse  e=[0 1 0 ]  Ts=0
  Sum2 : Sum  Commented=on  Inputs=|++
  Switch1 : Switch  Threshold=1  SaturateOnIntegerOverflow=off
  T1 : spsThreePhaseTransformerTwoWindingsLib/Three-Phase Transformer (Two Windings)  Winding1Connection=Delta (D1)  Winding2Connection=Yg  CoreType=Three single-phase transformers  SetSaturation=off  Hysteresis=off  DataFile='hysteresis'  SetInitialFlux=off  Measurements=None  UNITS=pu  NominalPower=[ 900E6 , 60 ]  Winding1=[ 20E3 , 1E-6 , 0.0]  Winding2=[ 230E3 , 1E-6 , 0.15 ]  Rm=1e4  Lm=1e4  L0=0.5  Saturation=[ 0,0 ; 0.0024,1.2 ; 1.0,1.52 ]  InitialFluxes=[ 0.8 , -0.8 , 0.7 ]  BreakLoop=off  DiscreteSolver=Trapezoidal iterative  DataType=off  TransfoNumber=1
  T2 : spsThreePhaseTransformerTwoWindingsLib/Three-Phase Transformer (Two Windings)  Winding1Connection=Delta (D1)  Winding2Connection=Yg  CoreType=Three single-phase transformers  SetSaturation=off  Hysteresis=off  DataFile='hysteresis'  SetInitialFlux=off  Measurements=None  UNITS=pu  NominalPower=[ 900E6 , 60 ]  Winding1=[ 20E3 , 1E-6 , 0.0 ]  Winding2=[ 230E3 , 1E-6 , 0.15 ]  Rm=1e4  Lm=1e4  L0=0.5  Saturation=[ 0,0 ; 0.0024,1.2 ; 1.0,1.52 ]  InitialFluxes=[ 0.8 , -0.8 , 0.7 ]  BreakLoop=off  DiscreteSolver=Trapezoidal iterative  DataType=off  TransfoNumber=1
  T3 : spsThreePhaseTransformerTwoWindingsLib/Three-Phase Transformer (Two Windings)  Winding1Connection=Delta (D1)  Winding2Connection=Yg  CoreType=Three single-phase transformers  SetSaturation=off  Hysteresis=off  DataFile='hysteresis'  SetInitialFlux=off  Measurements=None  UNITS=pu  NominalPower=[ 900E6 , 60 ]  Winding1=[ 20E3 , 1E-6 , 0.0]  Winding2=[ 230E3 , 1E-6 , 0.15 ]  Rm=1e4  Lm=1e4  L0=0.5  Saturation=[ 0,0 ; 0.0024,1.2 ; 1.0,1.52 ]  InitialFluxes=[ 0.8 , -0.8 , 0.7 ]  BreakLoop=off  DiscreteSolver=Trapezoidal iterative  DataType=off  TransfoNumber=1
  T4 : spsThreePhaseTransformerTwoWindingsLib/Three-Phase Transformer (Two Windings)  Winding1Connection=Delta (D1)  Winding2Connection=Yg  CoreType=Three single-phase transformers  SetSaturation=off  Hysteresis=off  DataFile='hysteresis'  SetInitialFlux=off  Measurements=None  UNITS=pu  NominalPower=[ 900E6 , 60 ]  Winding1=[ 20E3 , 1E-6 , 0.0 ]  Winding2=[ 230E3 , 1E-6 , 0.15]  Rm=1e4  Lm=1e4  L0=0.5  Saturation=[ 0,0 ; 0.0024,1.2 ; 1.0,1.52 ]  InitialFluxes=[ 0.8 , -0.8 , 0.7 ]  BreakLoop=off  DiscreteSolver=Trapezoidal iterative  DataType=off  TransfoNumber=1
  T5 : spsThreePhaseTransformerTwoWindingsLib/Three-Phase Transformer (Two Windings)  Commented=on  Winding1Connection=Yg  Winding2Connection=Yg  CoreType=Three single-phase transformers  SetSaturation=off  Hysteresis=off  DataFile='hysteresis'  SetInitialFlux=off  Measurements=None  UNITS=pu  NominalPower=[ 112E3 , 60 ]  Winding1=[ 142E3 , 1E-6 , 0.0 ]  Winding2=[ 230E3 , 1E-6 , 0.15 ]  Rm=500  Lm=500  L0=0.5  Saturation=[ 0,0 ; 0.0024,1.2 ; 1.0,1.52 ]  InitialFluxes=[ 0.8 , -0.8 , 0.7 ]  BreakLoop=off  DiscreteSolver=Trapezoidal iterative  DataType=off  TransfoNumber=1
  Three-Phase Transformer (Three Windings) : spsThreePhaseTransformerThreeWindingsLib/Three-Phase Transformer (Three Windings)  Commented=on  Winding1Connection=Yg  Winding2Connection=Yg  Winding3Connection=Delta (D1)  CoreType=Three single-phase transformers  SetSaturation=off  Hysteresis=off  DataFile='hysteresis'  SetInitialFlux=off  Measurements=None  UNITS=pu  NominalPower=[ 250e6 , 60 ]  Winding1=[ 735e3 , 0.002 , 0.08 ]  Winding2=[ 315e3 , 0.002 , 0.08 ]  Winding3=[ 315e3 , 0.002 , 0.08 ]  Rm=500  Lm=500  L0=0.5  Saturation=[ 0,0 ; 0.0024,1.2 ; 1.0,1.52 ]  InitialFluxes=[0.8 -0.8 0.7]  BreakLoop=off  DiscreteSolver=Trapezoidal iterative  DataType=off  TransfoNumber=1
      settings: LibrarySourceBlock=|
      | sps_lib/Power Grid Elements/Three-Phase
      | Transformer
      | (Three Windings)
  Three-Phase Source1 : spsThreePhaseSourceLib/Three-Phase Source  Commented=on  InternalConnection=Yg  VoltagePhases=off  Voltage=Vnom*0.995  PhaseAngle=0  Voltage_phases=[25e3 25e3 25e3]/sqrt(3)  PhaseAngles_phases=[0 -120 +120]  Frequency=60  NonIdealSource=on  SpecifyImpedance=on  Resistance=0.8929  Inductance=16.58e-3  ShortCircuitLevel=20e5  BaseVoltage=Vnom  XRratio=10  BusType=swing  Pref=10e3  Qref=0  Prefabc=[10e3, 10e3, 10e3]  Qrefabc=[0, 0, 0]  Qmin=-inf  Qmax=inf
  Toggle Switch{,1..5} (6 alike) : ToggleSwitchBlock  Commented=on  LabelPosition=Hide
  Utility-scale Solar Electrical Controller : Subsystem  Commented=on  mask(Renewable Energy Electrical Controller (REEC_B)){Trv=reec_Trv, Vdip=reec_Vdip, Vup=reec_Vup, dbd1=reec_dbd1, dbd2=reec_dbd2, Kqv=0, Iqhl=reec_Iqhl, Iqll=reec_Iqll, Tp=reec_Tp, Qmax=reec_Qmax, Qmin=reec_Qmin, Kqp=reec_Kqp, Kqi=reec_Kqi, Vmax=reec_Vmax, Vmin=reec_Vmin, Kvp=reec_Kvp, Kvi=reec_Kvi, Tiq=reec_Tiq, Tpord=reec_Tpord, Pmax=reec_Pmax, Pmin=reec_Pmin, dPmax=reec_dPmax, dPmin=reec_dPmin, Imax=reec_Imax}
      mask prompts: Trv "Trv - Terminal Bus Filter [s]"; Vdip "Vdip - Low Voltage Trigger [pu]"; Vup "Vup - High Voltage Trigger [pu]"; dbd1 "dbd1 - Overvoltage deadband [pu]"; dbd2 "dbd2 - Undervoltage deadband [pu]"; Kqv "Kqv - Reactive current injection gain [pu]"; Iqhl "Iqhl - Maximum current injection [pu]"; Iqll "Iqll - Minimum current injection [pu]"; Tp "Tp - Active Power Time Constant [s]"; Qmax "Qmax - Maximum reactive power [pu]"; Qmin "Qmin - Minimum reactive power [pu]"; Kqp "Kqp - Local Q regulator [pu]"; Kqi "Kqi - Local Q integrator gain [pu]"; Vmax "Vmax - Maximum inverter voltage [pu]"; Vmin "Vmin - Minium inverter terminal voltage [pu]"; Kvp "Kvp - Voltage Regulator Gain [pu]"; Kvi "Kvi - Voltage Integrator Gain [pu]"; Tiq "Tiq - Reactive Power Lag [s]"; Tpord "Tpord - Inverter Lag Time Constant [s]"; Pmax "Pmax - Maximum active power [pu]"; Pmin "Pmin - Minimum active power [pu]"; dPmax "dPmax - Power Up-ramp Limit [pu/s]"; dPmin "dPmin - Power Down-ramp Limit [pu/s]"; Imax "Imax - Maximum apparent current [pu]"
      mask help: REEC_B module, used to represent the Electrical Controls of the inverters. It acts on the active and reactive power reference from the REPC_A module, with feedback of terminal voltage and generator power output, and provides real and reactive current commands to the REGC_A module.
      mask Display: color('blue');disp('REEC_A')
  Utility-scale Solar Plant Controller : Subsystem  Commented=on  mask(Renewable Energy Plant Controller (REPC_A)){Tfltr=repc_Tfltr, Xc=repc_Xc, Rc=repc_Rc, Kc=repc_Kc, db1=repc_db1, emax=repc_emax, emin=repc_emin, Kp=repc_Kp, Ki=repc_Ki, Qmax=repc_Qmax, Qmin=repc_Qmin, Vfrz=repc_Vfrz, Tft=repc_Tft, Tfv=repc_Tfv, fdbd1=repc_fdbd1, fdbd2=repc_fdbd2, Ddn=repc_Ddn, Dup=repc_Dup, Tp=repc_Tp, femax=repc_femax, femin=repc_femin, Kpg=repc_Kpg, Kig=repc_Kig, Tlag=repc_Tlag, Pmax=repc_Pmax, Pmin=repc_Pmin}
      mask prompts: Tfltr "Tfltr - Voltage/Reactive Power Time Constants [s]"; Xc "Xc - Line drop compensation reactance [pu]"; Rc "Rc - Line drop compensation resistance [pu]"; Kc "Kc - Reactive droop [pu]"; db1 "db - Reactive power deadline [pu]"; emax "emax - Maximum Volt/VAR error [pu]"; emin "emin - Minimum Volt/VAR error [pu]"; Kp "Kp - Volt/VAR Propotional Gain [pu/pu]"; Ki "Ki - Volt/VAR Integral Gain [pu/pu-s]"; Qmax "Qmax - Max Plant Reactive Power [pu]"; Qmin "Qmin - Min Plant Reactive Power [pu]"; Vfrz "Vfrz - Voltage for Freezing Volt/VAR Integrator [pu]"; Tft "Tft - Q Lead Time Constant [s]"; Tfv "Tfv - Q Lag Time Constant [s]"; fdbd1 "fdbd1 - Overfrequency deadband for govenor [pu]"; fdbd2 "fdbd2 - Underfrequency deadband for govenor [pu]"; Ddn "Ddn - Down regulation droop [pu]"; Dup "Dup - Up regulation droop [pu]"; Tp "Tp - Active Power Filter Time Constant [s]"; femax "femax - Maximum Power Error [pu]"; femin "femin - Minimum Power Error [pu]"; Kpg "Kpg - Droop regulator gain [pu]"; Kig "Kig - Droop integral gain [pu]"; Tlag "Tlag - Plant Controller P output Lag [s]"; Pmax "Pmax - Maximum Plant Active Power [pu]"; Pmin "Pmin - Minimum Plant Active Power [pu]"
      mask help: REPC_A module, used to represent the Plant Controller. It processes voltage and reactive power output to emulate volt/var control at the plant level. It also processes frequency and active power output to emulate active power control. This module provides active reactive power command to the REEC_B module.
      mask Display: color('blue');disp('REPC_A')
  Vref : Constant  Commented=on  Value=0.9867
  Vref1 1 : Constant  Value=1.03+0.02
  Vref2 : Constant  Value=1.03
  W1 : ToWorkspace  VariableName=PB1  SampleTime=1/60
  W10 : ToWorkspace  VariableName=PL2  SampleTime=1/60
  W11 : ToWorkspace  VariableName=QL2  SampleTime=1/60
  W12 : ToWorkspace  VariableName=QB3  SampleTime=1/60
  W13 : ToWorkspace  VariableName=QB4  SampleTime=1/60
  W14 : ToWorkspace  VariableName=QB1  SampleTime=1/60
  W15 : ToWorkspace  VariableName=QB2  SampleTime=1/60
  W2 : ToWorkspace  Commented=on  VariableName=PB5  SampleTime=1/60
  W3 : ToWorkspace  VariableName=PB3  SampleTime=1/60
  W4 : ToWorkspace  VariableName=PB4  SampleTime=1/60
  W5 : ToWorkspace  VariableName=PB2  SampleTime=1/60
  W6 : ToWorkspace  Commented=on  VariableName=PB5Q  SampleTime=1/60
  W7 : ToWorkspace  VariableName=PL1  SampleTime=1/60
  W8 : ToWorkspace  Commented=on  VariableName=F5  SampleTime=1/60
  W9 : ToWorkspace  VariableName=QL1  SampleTime=1/60
  powergui : spspowerguiLib/powergui  Priority=1  SimulationMode=Phasor  SampleTime=50e-6  frequency=60  Iterations=500  frequencyindice=60  Pbase=100e6  ErrMax=1e-4  UnitsV=kV  UnitsW=MW  buscounter=0  FunctionMessages=off  echomessages=on  EnableUseOfTLC=off  CurrentSourceSwitches=off  DisableSnubberDevices=off  DisableRonSwitches=off  DisableVfSwitches=off  DisplayEquations=off  AutomaticDiscreteSolvers=off  SolverType=Tustin/Backward Euler (TBE)  Interpol=off  ExternalGateDelay=off  methode=off  Ts=100  x0status=blocks  SPID=on  SwTol=0  HookPort=off  NonlinearTolerance=0  nMaxIteration=15  ContinueOnMaxIteration=off  RestoreLinks=warning  ResistiveCurrentMeasurement=off  Frange=[0:2:500]  Ylog=off  Xlog=on  ShowGrid=off  save=off  variable=ZData  structure=0  ZoomFFT=off  StartTime=0.0  cycles=1  DisplayStyle=1  fundamental=60  FreqAxis=off  MaxFrequency=1000  frequencyindicesteady=1  RmsSteady=1  display=off
  to PU : Gain  Commented=on  Gain=1/Vnom
  to PU{1..2,4,6} (4 alike) : Gain  Commented=on  Gain=1/Pnom
  to PU3 : Gain  Commented=on  Gain=1/Vnom
  to PU5 : Gain  Commented=on  Gain=1/Fnom
  tag scope: INPSS=global, PB1=global, PB2=global, PB3=global, PB4=global, QB1=global, QB2=global, QB3=global, QB4=global
  wires:
  Renewable Grid-Connection/1(m) -> Goto/1, Selection/1(In1)
  Utility-scale Solar Plant Controller/1(Pext) -> Utility-scale Solar Electrical Controller/2(Pref)
  Bus Selector1/3 -> to PU2/1  "<Q>"
  Bus Selector1/1 -> to PU/1  "<V>"
  Bus Selector1/2 -> to PU1/1  "<P>"
  From/1 -> Bus Selector1/1
  to PU/1 -> Utility-scale Solar Electrical Controller/4(Vt)
  Utility-scale Solar Electrical Controller/1(Iq_cmd) -> Renewable Grid-Connection/1(Iq_cmd)  "Iq_cmd"
  Utility-scale Solar Electrical Controller/2(Ip_cmd) -> Renewable Grid-Connection/2(Ip_cmd)  "Ip_cmd"
  to PU1/1 -> Utility-scale Solar Electrical Controller/5(Pgen)  "P"
  to PU2/1 -> Utility-scale Solar Electrical Controller/6(Qgen)  "Q"
  Bus Selector2/3 -> to PU6/1  "<Q>"
  to PU6/1 -> Signal Conversion2/1
  Signal Conversion2/1 -> Bus Creator2/3  "Qbranch"
  Signal Conversion/1 -> Bus Creator2/1  "Freq"
  to PU3/1 -> Utility-scale Solar Plant Controller/4(Vreg)
  Bus Creator1/1 -> Utility-scale Solar Plant Controller/2(Refs)  "Refs"
  Signal Conversion1/1 -> Bus Creator2/2  "Pbranch"
  to PU5/1 -> Signal Conversion/1
  Constant13/1 -> Bus Creator1/2  "Fref"
  Bus Selector2/2 -> to PU4/1  "<P>"
  From2/1 -> Bus Selector3/1
  Pref/1 -> Bus Creator1/3, Goto1/1  "Pref"
  Bus Creator2/1 -> Utility-scale Solar Plant Controller/3(" Meas")  "Meas"
  Constant14/1 -> Bus Creator2/4  "Ibranch"
  Bus Selector2/1 -> to PU5/1  "<F>"
  Qref/1 -> Goto3/1, Bus Creator1/4  "Qref"
  From1/1 -> Bus Selector2/1
  to PU4/1 -> Signal Conversion1/1
  Bus Selector3/1 -> to PU3/1  "<V>"
  Utility-scale Solar Plant Controller/2(Qext) -> Utility-scale Solar Electrical Controller/3(Qref)
  Vref/1 -> Bus Creator1/1, Goto2/1  "Vref"
  Local and Plant Level Controller/1(Mode) -> Utility-scale Solar Plant Controller/1(Mode), Utility-scale Solar Electrical Controller/1(Mode)
  P/Q Priority/1 -> Local and Plant Level Controller/6(PQPriority)
  Plant-Level Control/1 -> Local and Plant Level Controller/5(PlantControl)
  Governor Response/1 -> Local and Plant Level Controller/4(FrqControl)
  PF Control/1 -> Local and Plant Level Controller/3(PFControl)
  Coordinated V/Q/1 -> Local and Plant Level Controller/2(QVControl)
  Q or V Control/1 -> Local and Plant Level Controller/1(QControl)
  Selection/1(Out1) -> Measurements/1
  Selection/2(<F>) -> W8/1, Measurements/2
  Selection/3(Out3) -> Measurements/3
  Selection/4(Out4) -> Measurements/4
  [Iabc_B1] -> 3-Phase Active & Reactive Power (Phasor Type)1/2
  [INPSS] -> "G3: Exciter, Turbine and Governor"/4(PSS), "G4: Exciter, Turbine and Governor"/4(PSS)
  Machine signals/1(d_theta1) -> Generators/1
  OFF/ON PSS/1 -> [INPSS]
  Constant/1 -> "G1: Exciter, Turbine and Governor"/2(Pref)
  System measurements/1(Vps) -> System/1
  G2/1 -> "G2: Exciter, Turbine and Governor"/1(m)
  System measurements/2(P_B7->B9) -> System/2
  Selector1/1 -> ->MW/1
  3-Phase Active & Reactive Power (Phasor Type)1/1 -> Selector1/1
  ->MW/1 -> [PB1], W1/1, Scope/1
  Machine signals/4(Vt) -> Generators/4
  G3/1 -> "G3: Exciter, Turbine and Governor"/1(m)
  Machine signals/2(dthetaT) -> Generators/2
  G1/1 -> "G1: Exciter, Turbine and Governor"/1(m)
  Machine signals/3(Pa) -> Scope10/1, Generators/3
  G4/1 -> "G4: Exciter, Turbine and Governor"/1(m)
  [INPSS] -> "G2: Exciter, Turbine and Governor"/4(PSS), "G1: Exciter, Turbine and Governor"/4(PSS)
  [Vabc_B1] -> 3-Phase Active & Reactive Power (Phasor Type)1/1
  Constant2/1 -> "G2: Exciter, Turbine and Governor"/2(Pref)
  Constant3/1 -> "G2: Exciter, Turbine and Governor"/3(Vref)
  Constant5/1 -> "G3: Exciter, Turbine and Governor"/2(Pref)
  Switch1/1 -> Scope13/1, "G3: Exciter, Turbine and Governor"/3(Vref)
  Constant7/1 -> "G4: Exciter, Turbine and Governor"/2(Pref)
  Constant6/1 -> "G4: Exciter, Turbine and Governor"/3(Vref)
  3-Phase Active & Reactive Power (Phasor Type)2/1 -> Selector2/1
  From8/1 -> 3-Phase Active & Reactive Power (Phasor Type)2/1
  From7/1 -> 3-Phase Active & Reactive Power (Phasor Type)2/2
  Selector2/1 -> ->MW1/1
  3-Phase Active & Reactive Power (Phasor Type)3/1 -> Selector3/1
  [Iabc_B3] -> 3-Phase Active & Reactive Power (Phasor Type)3/2
  Selector3/1 -> ->MW2/1
  ->MW2/1 -> [PB3], W3/1, Scope2/1
  [Vabc_B3] -> 3-Phase Active & Reactive Power (Phasor Type)3/1
  ->MW3/1 -> [PB4], W4/1, Scope3/1
  [Vabc_B4] -> 3-Phase Active & Reactive Power (Phasor Type)4/1
  Selector4/1 -> ->MW3/1
  3-Phase Active & Reactive Power (Phasor Type)4/1 -> Selector4/1
  [Iabc_B4] -> 3-Phase Active & Reactive Power (Phasor Type)4/2
  Selector5/1 -> ->MW4/1
  3-Phase Active & Reactive Power (Phasor Type)5/1 -> Selector5/1
  [Vabc_B7c] -> 3-Phase Active & Reactive Power (Phasor Type)5/1
  [Iabc_B7c] -> 3-Phase Active & Reactive Power (Phasor Type)5/2
  ->MW4/1 -> W7/1, Scope4/1
  Selector6/1 -> ->MW5/1
  3-Phase Active & Reactive Power (Phasor Type)6/1 -> Selector6/1
  [Vabc_B9c] -> 3-Phase Active & Reactive Power (Phasor Type)6/1
  [Iabc_B9c] -> 3-Phase Active & Reactive Power (Phasor Type)6/2
  ->MW5/1 -> W10/1, Scope5/1
  [Iabc_B7c] -> 3-Phase Active & Reactive Power (Phasor Type)7/2
  ->MW6/1 -> W9/1, Scope6/1
  [Vabc_B7c] -> 3-Phase Active & Reactive Power (Phasor Type)7/1
  3-Phase Active & Reactive Power (Phasor Type)7/1 -> Selector7/1
  Selector7/1 -> ->MW6/1
  3-Phase Active & Reactive Power (Phasor Type)8/1 -> Selector8/1
  [Iabc_B9c] -> 3-Phase Active & Reactive Power (Phasor Type)8/2
  [Vabc_B9c] -> 3-Phase Active & Reactive Power (Phasor Type)8/1
  Selector8/1 -> ->MW7/1
  ->MW7/1 -> W11/1, Scope7/1
  ->MW8/1 -> [PB2], W5/1, Scope8/1
  [Iabc_B2] -> 3-Phase Active & Reactive Power (Phasor Type)9/2
  Selector9/1 -> ->MW8/1
  3-Phase Active & Reactive Power (Phasor Type)9/1 -> Selector9/1
  [Vabc_B2] -> 3-Phase Active & Reactive Power (Phasor Type)9/1
  From24/1 -> 3-Phase Active & Reactive Power (Phasor Type)10/1
  From23/1 -> 3-Phase Active & Reactive Power (Phasor Type)10/2
  3-Phase Active & Reactive Power (Phasor Type)10/1 -> Selector10/1
  ->MW9/1 -> W6/1, Square/1, Scope9/1
  Selector10/1 -> ->MW9/1
  ->MW1/1 -> Square1/1, W2/1, Product/1, Scope1/1
  Square/1 -> Sum2/1
  Product/1 -> Display1/1
  Square1/1 -> Sum2/2
  Sqrt/1 -> Display/1, Product/2
  Sum2/1 -> Sqrt/1
  Stair Generator1/1 -> Switch1/2
  Vref2/1 -> Switch1/3
  Vref1 1/1 -> Switch1/1
  Selector11/1 -> ->MW10/1
  [Iabc_B8] -> Scope12/1, 3-Phase Active & Reactive Power (Phasor Type)11/2
  3-Phase Active & Reactive Power (Phasor Type)11/1 -> Selector11/1
  ->MW10/1 -> Scope11/1
  [Vabc_B8] -> 3-Phase Active & Reactive Power (Phasor Type)11/1
  "G1: Exciter, Turbine and Governor"/1(Pm) -> G1/1
  "G1: Exciter, Turbine and Governor"/2(Vf) -> G1/2
  "G2: Exciter, Turbine and Governor"/1(Pm) -> G2/1
  "G2: Exciter, Turbine and Governor"/2(Vf) -> G2/2
  "G4: Exciter, Turbine and Governor"/2(Vf) -> G4/2
  "G4: Exciter, Turbine and Governor"/1(Pm) -> G4/1
  "G3: Exciter, Turbine and Governor"/1(Pm) -> G3/1
  "G3: Exciter, Turbine and Governor"/2(Vf) -> G3/2
  Constant1/1 -> "G1: Exciter, Turbine and Governor"/3(Vref)
  3-Phase Active & Reactive Power (Phasor Type)12/1 -> Selector12/1
  [Iabc_B2] -> 3-Phase Active & Reactive Power (Phasor Type)12/2
  [Vabc_B2] -> 3-Phase Active & Reactive Power (Phasor Type)12/1
  Selector12/1 -> ->MW11/1
  Sequence Analyzer (Phasor Type)2/1 -> ->pu1/1
  ->pu1/1 -> Scope15/1
  [Vabc_B2] -> Sequence Analyzer (Phasor Type)2/1
  ->MW12/1 -> [QB3], W12/1, Scope16/1
  [Vabc_B3] -> 3-Phase Active & Reactive Power (Phasor Type)13/1
  Selector13/1 -> ->MW12/1
  3-Phase Active & Reactive Power (Phasor Type)13/1 -> Selector13/1
  [Iabc_B3] -> 3-Phase Active & Reactive Power (Phasor Type)13/2
  Selector15/1 -> ->MW14/1
  3-Phase Active & Reactive Power (Phasor Type)15/1 -> Selector15/1
  ->MW14/1 -> [QB1], W14/1, Scope18/1
  [Iabc_B1] -> 3-Phase Active & Reactive Power (Phasor Type)15/2
  [Vabc_B1] -> 3-Phase Active & Reactive Power (Phasor Type)15/1
  [Vabc_B1] -> Sequence Analyzer (Phasor Type)1/1
  Sequence Analyzer (Phasor Type)1/1 -> ->pu2/1
  ->pu2/1 -> Scope19/1
  3-Phase Active & Reactive Power (Phasor Type)14/1 -> Selector14/1
  [Iabc_B4] -> 3-Phase Active & Reactive Power (Phasor Type)14/2
  [Vabc_B4] -> 3-Phase Active & Reactive Power (Phasor Type)14/1
  ->MW13/1 -> [QB4], W13/1, Scope17/1
  Selector14/1 -> ->MW13/1
  ->pu3/1 -> Scope20/1
  [Vabc_B3] -> Sequence Analyzer (Phasor Type)3/1
  Sequence Analyzer (Phasor Type)3/1 -> ->pu3/1
  ->pu4/1 -> Scope21/1
  [Vabc_B4] -> Sequence Analyzer (Phasor Type)4/1
  Sequence Analyzer (Phasor Type)4/1 -> ->pu4/1
  ->MW11/1 -> [QB2], W15/1, Scope14/1
  connections:
  110 Km LT78/RConn2 -- 110 Km LT98/RConn2 -- 110 Km LT87/RConn2 -- 110 Km LT89/RConn2
  G2/RConn1 -- T2/LConn1 -- Bus*16*/LConn1
  110 Km LT98/LConn1 -- B6/LConn1 -- B9/LConn1 -- 110 Km LT89/LConn1
  10 Km LT910/LConn1 -- B4/RConn1 -- 25 Km LT1011/RConn1
  T3/LConn1 -- G3/RConn1 -- Bus*18*/LConn1
  T1/LConn1 -- G1/RConn1 -- Bus*14*/LConn1
  110 Km LT89/LConn2 -- 110 Km LT98/LConn2 -- B6/LConn2 -- B9/LConn2
  B9/LConn3 -- B6/LConn3 -- 110 Km LT98/LConn3 -- 110 Km LT89/LConn3
  10 Km LT910/LConn3 -- 25 Km LT1011/RConn3 -- B4/RConn3
  110 Km LT87/LConn2 -- B7/RConn2 -- 110 Km LT78/LConn2
  Bus*17*/LConn1 -- B3/LConn1 -- T3/RConn1
  110 Km LT87/LConn3 -- B7/RConn3 -- 110 Km LT78/LConn3
  G4/RConn1 -- T4/LConn1 -- Bus*20*/LConn1
  10 Km LT67/LConn2 -- B2/RConn2 -- 25 Km LT56/RConn2 -- B5/RConn2
  Bus*13*/LConn1 -- B1/LConn1 -- T1/RConn1
  10 Km LT910/LConn2 -- B4/RConn2 -- 25 Km LT1011/RConn2
  110 Km LT87/LConn1 -- B7/RConn1 -- 110 Km LT78/LConn1
  G2/RConn3 -- T2/LConn3
  B1/LConn2 -- T1/RConn2
  T3/LConn2 -- G3/RConn2
  T1/LConn3 -- G1/RConn3
  B1/RConn3 -- 25 Km LT56/LConn3
  B1/LConn3 -- T1/RConn3
  G4/RConn3 -- T4/LConn3
  G4/RConn2 -- T4/LConn2
  T3/LConn3 -- G3/RConn3
  B1/RConn2 -- 25 Km LT56/LConn2
  G2/RConn2 -- T2/LConn2
  T1/LConn2 -- G1/RConn2
  B1/RConn1 -- 25 Km LT56/LConn1
  10 Km LT67/LConn3 -- B5/RConn3 -- B2/RConn3 -- 25 Km LT56/RConn3
  10 Km LT67/LConn1 -- B5/RConn1 -- B2/RConn1 -- 25 Km LT56/RConn1
  Bus*22*/LConn1 -- C9 -350 Mvar/LConn1 -- B9c/RConn1 -- L9 1767 MW 100 Mvar/LConn1
  10 Km LT910/RConn2 -- B9c/LConn2 -- B9/RConn2
  B9/RConn3 -- 10 Km LT910/RConn3 -- B9c/LConn3
  C7 -200 Mvar/LConn3 -- B7c/RConn3 -- L7 967 MW 100 Mvar/LConn3
  B7/LConn2 -- 10 Km LT67/RConn2 -- B7c/LConn2
  C7 -200 Mvar/LConn1 -- Bus*21*/LConn1 -- B7c/RConn1 -- L7 967 MW 100 Mvar/LConn1
  B5/LConn1 -- Renewable Grid-Connection/RConn1 -- Load Flow Bus2/LConn1
  B4/LConn3 -- T4/RConn3
  T3/RConn3 -- B3/LConn3
  B3/LConn2 -- T3/RConn2
  B3/RConn1 -- 25 Km LT1011/LConn1
  25 Km LT1011/LConn2 -- B3/RConn2
  25 Km LT1011/LConn3 -- B3/RConn3
  T4/RConn2 -- B4/LConn2
  T4/RConn1 -- B4/LConn1 -- Bus*19*/LConn1
  Shunt/LConn1 -- Three-Phase Source1/RConn1
  Shunt/LConn3 -- Three-Phase Source1/RConn3
  Shunt/RConn1 -- Shunt/RConn2 -- Ground/LConn1 -- Shunt/RConn3
  Shunt/LConn2 -- Three-Phase Source1/RConn2
  B5/LConn2 -- Renewable Grid-Connection/RConn2
  Renewable Grid-Connection/RConn3 -- B5/LConn3
  B7/LConn1 -- B7c/LConn1 -- 10 Km LT67/RConn1
  C7 -200 Mvar/LConn2 -- B7c/RConn2 -- L7 967 MW 100 Mvar/LConn2
  B7/LConn3 -- B7c/LConn3 -- 10 Km LT67/RConn3
  L9 1767 MW 100 Mvar/LConn2 -- B9c/RConn2 -- C9 -350 Mvar/LConn2
  C9 -350 Mvar/LConn3 -- B9c/RConn3 -- L9 1767 MW 100 Mvar/LConn3
  B9/RConn1 -- 10 Km LT910/RConn1 -- B9c/LConn1
  B2/LConn3 -- T2/RConn3
  B2/LConn2 -- T2/RConn2
  T2/RConn1 -- B2/LConn1 -- Load Flow Bus/LConn1
  110 Km LT78/RConn3 -- 110 Km LT89/RConn3 -- 110 Km LT98/RConn3 -- 110 Km LT87/RConn3
  Fault/LConn2 -- B6/RConn2
  Fault/LConn3 -- B6/RConn3
  Fault/LConn1 -- B6/RConn1
  110 Km LT78/RConn1 -- 110 Km LT98/RConn1 -- 110 Km LT87/RConn1 -- 110 Km LT89/RConn1
